simulink model "Controller"  (R2018b)
settings: configuration reference "control_config" (kept outside this file)
values from neighbouring files (symbols this model uses):
  CONTROL_EXPORT = Simulink.Parameter(CONTROL_EXPORT_VALUE)    [controller_model_init.m]
  CONTROL_PARAM = Simulink.Parameter(CONTROL_PARAM_VALUE)    [controller_model_init.m]
undefined symbols (not defined in the file or in its folder): actuator_cmd, CONTROL_CONST, ControlMode, DiscIntNeverNeededParam, timestamp, VehicleStatus
libraries: simulink x27, FMT_Model_Lib x7
(part 1 of 3)
settings Model: Creator=jc  LastModifiedBy=zouji
settings ConfigSetRef: SourceLocation=Base Workspace

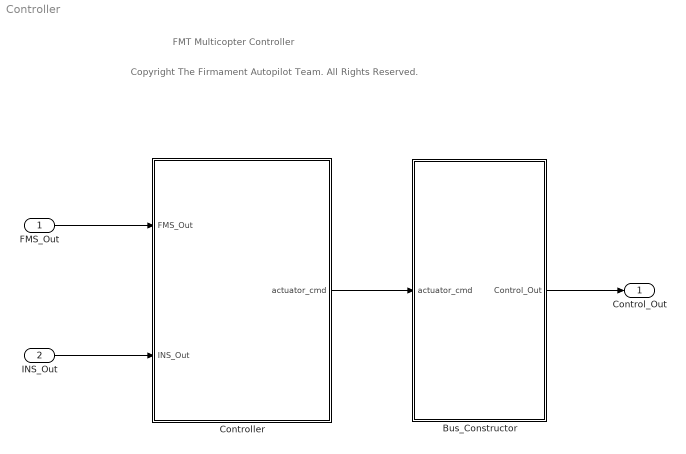
== system Controller ==
  note: Copyright The Firmament Autopilot Team. All Rights Reserved.
  note: FMT Multicopter Controller
  FMS_Out : Inport  OutDataTypeStr=Bus: FMS_Out_Bus
  INS_Out : Inport  Port=2  OutDataTypeStr=Bus: INS_Out_Bus
  Bus_Constructor : Subsystem
  Controller : Subsystem
  Control_Out : Outport  OutDataTypeStr=Bus: Control_Out_Bus
  wires:
  FMS_Out/1 -> Controller/1(FMS_Out)
  INS_Out/1 -> Controller/2(INS_Out)
  Controller/1(actuator_cmd) -> Bus_Constructor/1(actuator_cmd)
  Bus_Constructor/1(Control_Out) -> Control_Out/1

== system Controller/Bus_Constructor ==
  actuator_cmd : Inport
  Bus Assignment : BusAssignment  AssignedSignals=actuator_cmd,timestamp
  Constant : Constant  Value=0  OutDataTypeStr=Bus: Control_Out_Bus
  timestamp : Subsystem  mask{sample_time=CONTROL_EXPORT.period}
      mask prompts: sample_time "sample time (ms)"
  Control_Out : Outport
  wires:
  actuator_cmd/1 -> Bus Assignment/2
  Constant/1 -> Bus Assignment/1
  Bus Assignment/1 -> Control_Out/1
  timestamp/1(timestamp_ms) -> Bus Assignment/3

== system Controller/Controller ==
  FMS_Out : Inport
  INS_Out : Inport  Port=2
  Control_Allocation : Subsystem  Variant=on
      settings: GeneratePreprocessorConditionals=on
  Horizontal_Control : Subsystem
  Vertical_Control : Subsystem
  actuator_cmd : Outport
  wires:
  FMS_Out/1 -> Vertical_Control/1(FMS_Out), Control_Allocation/1(FMS_Out), Horizontal_Control/1(FMS_Out)
  INS_Out/1 -> Vertical_Control/2(INS_Out), Horizontal_Control/2(INS_Out)
  Horizontal_Control/1(torque_cmd_B) -> Control_Allocation/2(torque_cmd_B)  "torque_cmd_B"
  Vertical_Control/1(throttle_cmd_B) -> Control_Allocation/3(throttle_cmd_B)  "throttle_cmd_B"
  Control_Allocation/1(actuator_cmd) -> actuator_cmd/1

== system Controller/Bus_Constructor/timestamp ==
  Constant : Constant  Value=sample_time
  Data Type Conversion : DataTypeConversion  OutDataTypeStr=uint32
  Discrete-Time Integrator : DiscreteIntegrator  IntegratorMethod=Accumulation: Forward Euler  SampleTime=-1  ICPrevOutput=DiscIntNeverNeededParam  ICPrevScaledInput=DiscIntNeverNeededParam
  timestamp_ms : Outport
  wires:
  Discrete-Time Integrator/1 -> Data Type Conversion/1
  Constant/1 -> Discrete-Time Integrator/1
  Data Type Conversion/1 -> timestamp_ms/1

== system Controller/Controller/Control_Allocation ==
  note: 1) Add Subsystem or Model blocks as valid variant choices.
      | 2) You cannot connect blocks at this level. At simulation, connectivity is automatically
      | determined, based on the active variant and port name matching.
  FMS_Out : Inport
  torque_cmd_B : Inport  Port=2
  throttle_cmd_B : Inport  Port=3
  Coxial_Hexacopter_x : Subsystem  TreatAsAtomicUnit=on  VariantControl=AIRFRAME==6
      mask Display: image('.\figures\cox_hexa_x.png');
  Coxial_Quadcopter_x : Subsystem  TreatAsAtomicUnit=on  VariantControl=AIRFRAME==3
      mask Display: image('.\figures\cox_quad_x.png');
  Hexacopter_+ : Subsystem  TreatAsAtomicUnit=on  VariantControl=AIRFRAME==5
      mask Display: image('.\figures\hexa_+.png');
  Hexacopter_x : Subsystem  TreatAsAtomicUnit=on  VariantControl=AIRFRAME==4
      mask Display: image('.\figures\hexa_x.png');
  Octocopter_+ : Subsystem  TreatAsAtomicUnit=on  VariantControl=AIRFRAME==8
      mask Display: image('.\figures\octo_+.png');
  Octocopter_x : Subsystem  TreatAsAtomicUnit=on  VariantControl=AIRFRAME==7
      mask Display: image('.\figures\octo_x.png');
  Quadcopter_+ : Subsystem  TreatAsAtomicUnit=on  VariantControl=AIRFRAME==2
      mask Display: image('.\figures\quad_+.png');
  Quadcopter_x : Subsystem  TreatAsAtomicUnit=on  VariantControl=AIRFRAME==1
      mask Display: image('.\figures\quad_x.png');
  actuator_cmd : Outport

== system Controller/Controller/Horizontal_Control ==
  FMS_Out : Inport
  INS_Out : Inport  Port=2
  Attitude_Controller : Subsystem
  Bus Selector : BusSelector  OutputSignals=ctrl_mode
  Compare To Constant : simulink/Logic and Bit Operations/Compare To Constant  relop=>=  const=uint8(ControlMode.POSCTL)  OutDataTypeStr=boolean
  Velocity_Controller : Subsystem
  torque_cmd_B : Outport
  wires:
  Attitude_Controller/1(rate_dot_cmd_B) -> torque_cmd_B/1
  FMS_Out/1 -> Bus Selector/1, Attitude_Controller/2(FMS_Out), Velocity_Controller/1(FMS_Out)
  INS_Out/1 -> Velocity_Controller/2(INS_Out), Attitude_Controller/3(INS_Out)
  Velocity_Controller/1(att_cmd_B_rad) -> Attitude_Controller/1(att_cmd_B_rad)
  Bus Selector/1 -> Compare To Constant/1  "<ctrl_mode>"
  Compare To Constant/1 -> Velocity_Controller/Enable

== system Controller/Controller/Vertical_Control ==
  FMS_Out : Inport
  INS_Out : Inport  Port=2
  Bus Selector : BusSelector  OutputSignals=ctrl_mode
  Bus Selector1 : BusSelector  OutputSignals=status
  Compare To Constant : simulink/Logic and Bit Operations/Compare To Constant  relop=>=  const=uint8(ControlMode.ALTCTL)  OutDataTypeStr=boolean
  Delay : Delay  DelayLength=1  InitialCondition=uint8(VehicleStatus.Disarm)
  Signal_Select : Subsystem
  Veloxity_Z_Controller : Subsystem
  throttle_cmd_B : Outport
  wires:
  INS_Out/1 -> Veloxity_Z_Controller/3(INS_Out)
  Veloxity_Z_Controller/1(throttle_cmd) -> Signal_Select/2(throttle_cmd_in)
  FMS_Out/1 -> Bus Selector1/1, Bus Selector/1, Signal_Select/1(FMS_Out), Veloxity_Z_Controller/1(FMS_Out)
  Bus Selector/1 -> Compare To Constant/1  "<ctrl_mode>"
  Compare To Constant/1 -> Veloxity_Z_Controller/Enable
  Bus Selector1/1 -> Delay/1  "<status>"
  Delay/1 -> Veloxity_Z_Controller/2(prev_status)
  Signal_Select/1(throttle_cmd) -> throttle_cmd_B/1

== system Controller/Controller/Control_Allocation/Coxial_Hexacopter_x ==
  FMS_Out : Inport
  torque_cmd_B : Inport  Port=2
  throttle_cmd_B : Inport  Port=3
  Bus Selector : BusSelector  OutputSignals=status
  Effective_Matrix : Constant  Value=[-1/2 0 -1/2;1/2 0 1/2;(sqrt(2)-1)/2 sqrt(6)/6 -1/2;-(sqrt(2)-1)/2 -sqrt(6)/6 1/2;-(sqrt(2)-1)/2 sqrt(6)/6 1/2;(sqrt(2)-1)/2 -sqrt(6)/6 -1/2;-1/2 0 1/2;1/2 0 -1/2;(sqrt(2)-1)/2 sqrt(6)/6 1/2;-(sqrt(2)-1)/2 -sqrt(6)/6 -1/2;-(sqrt(2)-1)/2 sqrt(6)/6 -1/2;(sqrt(2)-1)/2 -sqrt(6)/6 1/2]  OutDataTypeStr=single
  Roll_Pitch_Remix : Subsystem  mask{up_lim=0.9, lo_lim=0.1}
      mask prompts: up_lim "Upper Limit"; lo_lim "Lower Limit"
  Saturation1 : Saturate  UpperLimit=1  LowerLimit=-1
  Saturation2 : Saturate  UpperLimit=1  LowerLimit=0
  Yaw_Remix : Subsystem  mask{up_lim=0.9, lo_lim=0.1}
      mask prompts: up_lim "Upper Limit"; lo_lim "Lower Limit"
  actuator_cmd_routing : Subsystem
  actuator_cmd : Outport
  wires:
  Effective_Matrix/1 -> Roll_Pitch_Remix/1(Effective_Matrix), Yaw_Remix/1(Effective_Matrix)
  throttle_cmd_B/1 -> Saturation2/1
  torque_cmd_B/1 -> Saturation1/1
  Bus Selector/1 -> actuator_cmd_routing/2(status)  "<status>"
  Saturation1/1 -> Yaw_Remix/2(torque_cmd), Roll_Pitch_Remix/2(torque_cmd)
  Roll_Pitch_Remix/1(pq_remix_throttle) -> Yaw_Remix/3(pq_remix)
  Yaw_Remix/1(pqr_remix_throttle) -> actuator_cmd_routing/1(throttle_cmd)
  actuator_cmd_routing/1(actuator_cmd) -> actuator_cmd/1
  FMS_Out/1 -> Bus Selector/1
  Saturation2/1 -> Roll_Pitch_Remix/3(throttle_cmd)

== system Controller/Controller/Control_Allocation/Coxial_Quadcopter_x ==
  FMS_Out : Inport
  torque_cmd_B : Inport  Port=2
  throttle_cmd_B : Inport  Port=3
  Bus Selector : BusSelector  OutputSignals=status
  Effective_Matrix : Constant  Value=[-1/2 1/2 1/2;1/2 1/2 -1/2;1/2 -1/2 1/2;-1/2 -1/2 -1/2;1/2 1/2 1/2;-1/2 1/2 -1/2;-1/2 -1/2 1/2;1/2 -1/2 -1/2]  OutDataTypeStr=single
  Roll_Pitch_Remix : Subsystem  mask{up_lim=0.9, lo_lim=0.1}
      mask prompts: up_lim "Upper Limit"; lo_lim "Lower Limit"
  Saturation1 : Saturate  UpperLimit=1  LowerLimit=-1
  Saturation2 : Saturate  UpperLimit=1  LowerLimit=0
  Yaw_Remix : Subsystem  mask{up_lim=0.9, lo_lim=0.1}
      mask prompts: up_lim "Upper Limit"; lo_lim "Lower Limit"
  actuator_cmd_routing : Subsystem
  actuator_cmd : Outport
  wires:
  Roll_Pitch_Remix/1(pq_remix_throttle) -> Yaw_Remix/3(pq_remix)
  Effective_Matrix/1 -> Yaw_Remix/1(Effective_Matrix), Roll_Pitch_Remix/1(Effective_Matrix)
  torque_cmd_B/1 -> Saturation1/1
  throttle_cmd_B/1 -> Saturation2/1
  FMS_Out/1 -> Bus Selector/1
  Saturation1/1 -> Yaw_Remix/2(torque_cmd), Roll_Pitch_Remix/2(torque_cmd)
  Saturation2/1 -> Roll_Pitch_Remix/3(throttle_cmd)
  Yaw_Remix/1(pqr_remix_throttle) -> actuator_cmd_routing/1(throttle_cmd)
  actuator_cmd_routing/1(actuator_cmd) -> actuator_cmd/1
  Bus Selector/1 -> actuator_cmd_routing/2(status)  "<status>"

== system Controller/Controller/Control_Allocation/Hexacopter_+ ==
  FMS_Out : Inport
  torque_cmd_B : Inport  Port=2
  throttle_cmd_B : Inport  Port=3
  Bus Selector : BusSelector  OutputSignals=status
  Effective_Matrix : Constant  Value=[0 1/2 -1/2;0 -1/2 1/2;sqrt(6)/6 -(sqrt(2)-1)/2 -1/2;-sqrt(6)/6 (sqrt(2)-1)/2 1/2;sqrt(6)/6 (sqrt(2)-1)/2 1/2;-sqrt(6)/6 -(sqrt(2)-1)/2 -1/2]  OutDataTypeStr=single
  Roll_Pitch_Remix : Subsystem  mask{up_lim=0.9, lo_lim=0.1}
      mask prompts: up_lim "Upper Limit"; lo_lim "Lower Limit"
  Saturation1 : Saturate  UpperLimit=1  LowerLimit=-1
  Saturation2 : Saturate  UpperLimit=1  LowerLimit=0
  Yaw_Remix : Subsystem  mask{up_lim=0.9, lo_lim=0.1}
      mask prompts: up_lim "Upper Limit"; lo_lim "Lower Limit"
  actuator_cmd_routing : Subsystem
  actuator_cmd : Outport
  wires:
  Saturation1/1 -> Yaw_Remix/2(torque_cmd), Roll_Pitch_Remix/2(torque_cmd)
  Effective_Matrix/1 -> Roll_Pitch_Remix/1(Effective_Matrix), Yaw_Remix/1(Effective_Matrix)
  Saturation2/1 -> Roll_Pitch_Remix/3(throttle_cmd)
  throttle_cmd_B/1 -> Saturation2/1
  actuator_cmd_routing/1(actuator_cmd) -> actuator_cmd/1
  Bus Selector/1 -> actuator_cmd_routing/2(status)  "<status>"
  Roll_Pitch_Remix/1(pq_remix_throttle) -> Yaw_Remix/3(pq_remix)
  FMS_Out/1 -> Bus Selector/1
  Yaw_Remix/1(pqr_remix_throttle) -> actuator_cmd_routing/1(throttle_cmd)
  torque_cmd_B/1 -> Saturation1/1

== system Controller/Controller/Control_Allocation/Hexacopter_x ==
  FMS_Out : Inport
  torque_cmd_B : Inport  Port=2
  throttle_cmd_B : Inport  Port=3
  Bus Selector : BusSelector  OutputSignals=status
  Effective_Matrix : Constant  Value=[-1/2 0 -1/2;1/2 0 1/2;(sqrt(2)-1)/2 sqrt(6)/6 -1/2;-(sqrt(2)-1)/2 -sqrt(6)/6 1/2;-(sqrt(2)-1)/2 sqrt(6)/6 1/2;(sqrt(2)-1)/2 -sqrt(6)/6 -1/2]  OutDataTypeStr=single
  Roll_Pitch_Remix : Subsystem  mask{up_lim=0.9, lo_lim=0.1}
      mask prompts: up_lim "Upper Limit"; lo_lim "Lower Limit"
  Saturation1 : Saturate  UpperLimit=1  LowerLimit=-1
  Saturation2 : Saturate  UpperLimit=1  LowerLimit=0
  Yaw_Remix : Subsystem  mask{up_lim=0.9, lo_lim=0.1}
      mask prompts: up_lim "Upper Limit"; lo_lim "Lower Limit"
  actuator_cmd_routing : Subsystem
  actuator_cmd : Outport
  wires:
  throttle_cmd_B/1 -> Saturation2/1
  Saturation1/1 -> Yaw_Remix/2(torque_cmd), Roll_Pitch_Remix/2(torque_cmd)
  FMS_Out/1 -> Bus Selector/1
  Bus Selector/1 -> actuator_cmd_routing/2(status)  "<status>"
  Roll_Pitch_Remix/1(pq_remix_throttle) -> Yaw_Remix/3(pq_remix)
  Saturation2/1 -> Roll_Pitch_Remix/3(throttle_cmd)
  Yaw_Remix/1(pqr_remix_throttle) -> actuator_cmd_routing/1(throttle_cmd)
  Effective_Matrix/1 -> Yaw_Remix/1(Effective_Matrix), Roll_Pitch_Remix/1(Effective_Matrix)
  actuator_cmd_routing/1(actuator_cmd) -> actuator_cmd/1
  torque_cmd_B/1 -> Saturation1/1

== system Controller/Controller/Control_Allocation/Octocopter_+ ==
  FMS_Out : Inport
  torque_cmd_B : Inport  Port=2
  throttle_cmd_B : Inport  Port=3
  Bus Selector : BusSelector  OutputSignals=status
  Effective_Matrix : Constant  Value=[0 0.5 -0.5;0 -0.5 -0.5;-0.146 0.146 0.5;-0.146 -0.146 0.5;0.146 0.146 0.5;0.146 -0.146 0.5;0.5 0 -0.5;-0.5 0 -0.5]  OutDataTypeStr=single
  Roll_Pitch_Remix : Subsystem  mask{up_lim=0.9, lo_lim=0.1}
      mask prompts: up_lim "Upper Limit"; lo_lim "Lower Limit"
  Saturation1 : Saturate  UpperLimit=1  LowerLimit=-1
  Saturation2 : Saturate  UpperLimit=1  LowerLimit=0
  Yaw_Remix : Subsystem  mask{up_lim=0.9, lo_lim=0.1}
      mask prompts: up_lim "Upper Limit"; lo_lim "Lower Limit"
  actuator_cmd_routing : Subsystem
  actuator_cmd : Outport
  wires:
  throttle_cmd_B/1 -> Saturation2/1
  Saturation2/1 -> Roll_Pitch_Remix/3(throttle_cmd)
  actuator_cmd_routing/1(actuator_cmd) -> actuator_cmd/1
  Roll_Pitch_Remix/1(pq_remix_throttle) -> Yaw_Remix/3(pq_remix)
  Effective_Matrix/1 -> Roll_Pitch_Remix/1(Effective_Matrix), Yaw_Remix/1(Effective_Matrix)
  Yaw_Remix/1(pqr_remix_throttle) -> actuator_cmd_routing/1(throttle_cmd)
  Bus Selector/1 -> actuator_cmd_routing/2(status)  "<status>"
  Saturation1/1 -> Yaw_Remix/2(torque_cmd), Roll_Pitch_Remix/2(torque_cmd)
  torque_cmd_B/1 -> Saturation1/1
  FMS_Out/1 -> Bus Selector/1

== system Controller/Controller/Control_Allocation/Octocopter_x ==
  FMS_Out : Inport
  torque_cmd_B : Inport  Port=2
  throttle_cmd_B : Inport  Port=3
  Bus Selector : BusSelector  OutputSignals=status
  Effective_Matrix : Constant  Value=[-0.15 0.5 -0.5;0.15 -0.5 -0.5;-0.5 0.15 0.5;-0.15 -0.5 0.5;0.15 0.5 0.5;0.5 -0.15 0.5;0.5 0.15 -0.5;-0.5 -0.15 -0.5]  OutDataTypeStr=single
  Roll_Pitch_Remix : Subsystem  mask{up_lim=0.9, lo_lim=0.1}
      mask prompts: up_lim "Upper Limit"; lo_lim "Lower Limit"
  Saturation1 : Saturate  UpperLimit=1  LowerLimit=-1
  Saturation2 : Saturate  UpperLimit=1  LowerLimit=0
  Yaw_Remix : Subsystem  mask{up_lim=0.9, lo_lim=0.1}
      mask prompts: up_lim "Upper Limit"; lo_lim "Lower Limit"
  actuator_cmd_routing : Subsystem
  actuator_cmd : Outport
  wires:
  torque_cmd_B/1 -> Saturation1/1
  Bus Selector/1 -> actuator_cmd_routing/2(status)  "<status>"
  Yaw_Remix/1(pqr_remix_throttle) -> actuator_cmd_routing/1(throttle_cmd)
  Saturation2/1 -> Roll_Pitch_Remix/3(throttle_cmd)
  Saturation1/1 -> Yaw_Remix/2(torque_cmd), Roll_Pitch_Remix/2(torque_cmd)
  FMS_Out/1 -> Bus Selector/1
  Roll_Pitch_Remix/1(pq_remix_throttle) -> Yaw_Remix/3(pq_remix)
  actuator_cmd_routing/1(actuator_cmd) -> actuator_cmd/1
  throttle_cmd_B/1 -> Saturation2/1
  Effective_Matrix/1 -> Roll_Pitch_Remix/1(Effective_Matrix), Yaw_Remix/1(Effective_Matrix)

== system Controller/Controller/Control_Allocation/Quadcopter_+ ==
  FMS_Out : Inport
  torque_cmd_B : Inport  Port=2
  throttle_cmd_B : Inport  Port=3
  Bus Selector : BusSelector  OutputSignals=status
  Effective_Matrix : Constant  Value=[-1/2 0 1/2;1/2 0 1/2;0 1/2 -1/2;0 -1/2 -1/2]  OutDataTypeStr=single
  Roll_Pitch_Remix : Subsystem  mask{up_lim=0.9, lo_lim=0.1}
      mask prompts: up_lim "Upper Limit"; lo_lim "Lower Limit"
  Saturation1 : Saturate  UpperLimit=1  LowerLimit=-1
  Saturation2 : Saturate  UpperLimit=1  LowerLimit=0
  Yaw_Remix : Subsystem  mask{up_lim=0.9, lo_lim=0.1}
      mask prompts: up_lim "Upper Limit"; lo_lim "Lower Limit"
  actuator_cmd_routing : Subsystem
  actuator_cmd : Outport
  wires:
  Effective_Matrix/1 -> Yaw_Remix/1(Effective_Matrix), Roll_Pitch_Remix/1(Effective_Matrix)
  Roll_Pitch_Remix/1(pq_remix_throttle) -> Yaw_Remix/3(pq_remix)
  torque_cmd_B/1 -> Saturation1/1
  Yaw_Remix/1(pqr_remix_throttle) -> actuator_cmd_routing/1(throttle_cmd)
  Saturation1/1 -> Yaw_Remix/2(torque_cmd), Roll_Pitch_Remix/2(torque_cmd)
  actuator_cmd_routing/1(actuator_cmd) -> actuator_cmd/1
  Saturation2/1 -> Roll_Pitch_Remix/3(throttle_cmd)
  throttle_cmd_B/1 -> Saturation2/1
  FMS_Out/1 -> Bus Selector/1
  Bus Selector/1 -> actuator_cmd_routing/2(status)  "<status>"

== system Controller/Controller/Control_Allocation/Quadcopter_x ==
  FMS_Out : Inport
  torque_cmd_B : Inport  Port=2
  throttle_cmd_B : Inport  Port=3
  Bus Selector : BusSelector  OutputSignals=status
  Effective_Matrix : Constant  Value=[-1/2 1/2 1/2;1/2 -1/2 1/2;1/2 1/2 -1/2;-1/2 -1/2 -1/2]  OutDataTypeStr=single
  Roll_Pitch_Remix : Subsystem  mask{up_lim=0.9, lo_lim=0.1}
      mask prompts: up_lim "Upper Limit"; lo_lim "Lower Limit"
  Saturation1 : Saturate  UpperLimit=1  LowerLimit=-1
  Saturation2 : Saturate  UpperLimit=1  LowerLimit=0
  Yaw_Remix : Subsystem  mask{up_lim=0.9, lo_lim=0.1}
      mask prompts: up_lim "Upper Limit"; lo_lim "Lower Limit"
  actuator_cmd_routing : Subsystem
  actuator_cmd : Outport
  wires:
  Effective_Matrix/1 -> Yaw_Remix/1(Effective_Matrix), Roll_Pitch_Remix/1(Effective_Matrix)
  Saturation1/1 -> Yaw_Remix/2(torque_cmd), Roll_Pitch_Remix/2(torque_cmd)
  Roll_Pitch_Remix/1(pq_remix_throttle) -> Yaw_Remix/3(pq_remix)
  Bus Selector/1 -> actuator_cmd_routing/2(status)  "<status>"
  torque_cmd_B/1 -> Saturation1/1
  Yaw_Remix/1(pqr_remix_throttle) -> actuator_cmd_routing/1(throttle_cmd)
  throttle_cmd_B/1 -> Saturation2/1
  FMS_Out/1 -> Bus Selector/1
  actuator_cmd_routing/1(actuator_cmd) -> actuator_cmd/1
  Saturation2/1 -> Roll_Pitch_Remix/3(throttle_cmd)

== system Controller/Controller/Horizontal_Control/Attitude_Controller ==
  att_cmd_B_rad : Inport
  FMS_Out : Inport  Port=2
  INS_Out : Inport  Port=3
  Inner_Loop : Subsystem
  Outter_Loop : Subsystem
  rate_dot_cmd_B : Outport
  wires:
  INS_Out/1 -> Inner_Loop/2(INS_Out), Outter_Loop/2(INS_Out)
  FMS_Out/1 -> Inner_Loop/3(FMS_Out), Outter_Loop/3(FMS_Out)
  att_cmd_B_rad/1 -> Outter_Loop/1(att_cmd_rad)
  Outter_Loop/1(euler_rate_cmd_radPs) -> Inner_Loop/1(euler_rate_cmd_radPs)
  Inner_Loop/1(rate_dot_cmd_B) -> rate_dot_cmd_B/1

== system Controller/Controller/Horizontal_Control/Velocity_Controller ==
  FMS_Out : Inport
  INS_Out : Inport  Port=2
  Enable : EnablePort  StatesWhenEnabling=reset
  Accel_to_Attitude_CMD : Subsystem
  Bus Selector : BusSelector  OutputSignals=reset
  Error : Subsystem
  PID_Controller : Subsystem
  Signal_Select : Subsystem
  att_cmd_B_rad : Outport
  wires:
  FMS_Out/1 -> Signal_Select/2(FMS_Out), Error/2(FMS_Out), Bus Selector/1
  PID_Controller/1(accel_cmd_C) -> Signal_Select/1(acc_cmd_in)  "accel_cmd_C_mPs2"
  INS_Out/1 -> Error/1(INS_Out)
  Error/1(uv_err_C_mPs) -> PID_Controller/1(uv_err_C_mPs)
  Accel_to_Attitude_CMD/1(att_cmd_B_rad) -> att_cmd_B_rad/1
  Bus Selector/1 -> PID_Controller/2(reset)  "<reset>"
  Signal_Select/1(acc_cmd_out) -> Accel_to_Attitude_CMD/1(accel_cmd_C_mPs2)

== system Controller/Controller/Vertical_Control/Signal_Select ==
  FMS_Out : Inport
  throttle_cmd_in : Inport  Port=2
  Bias : Bias  Bias=-1
  Bus Selector1 : BusSelector  OutputSignals=throttle_cmd,ctrl_mode
  Compare To Constant : simulink/Logic and Bit Operations/Compare To Constant  relop=<=  const=uint8(ControlMode.Stabilize)  OutDataTypeStr=boolean
  Compare To Constant1 : simulink/Logic and Bit Operations/Compare To Constant  relop===  const=uint8(ControlMode.Offboard)  OutDataTypeStr=boolean
  Gain : Gain  Gain=1/1000  OutDataTypeStr=single
  Offboard_Signal_Select : Subsystem
  Switch : Switch  Criteria=u2 > Threshold
  Switch1 : Switch  Criteria=u2 > Threshold
  throttle_cmd : Outport
  wires:
  FMS_Out/1 -> Offboard_Signal_Select/1(FMS_Out), Bus Selector1/1
  Bus Selector1/1 -> Gain/1  "<throttle_cmd>"
  Bus Selector1/2 -> Compare To Constant/1, Compare To Constant1/1  "<ctrl_mode>"
  Switch/1 -> throttle_cmd/1
  Compare To Constant/1 -> Switch/2
  throttle_cmd_in/1 -> Offboard_Signal_Select/2(throttle_cmd_in), Switch1/3
  Compare To Constant1/1 -> Switch1/2
  Switch1/1 -> Switch/3
  Offboard_Signal_Select/1(throttle_cmd_out) -> Switch1/1
  Gain/1 -> Bias/1
  Bias/1 -> Switch/1

== system Controller/Controller/Vertical_Control/Veloxity_Z_Controller ==
  FMS_Out : Inport
  prev_status : Inport  Port=2
  INS_Out : Inport  Port=3
  Enable : EnablePort  StatesWhenEnabling=reset
  Boosted_Throttle : Subsystem
  Bus Selector : BusSelector  OutputSignals=reset
  Error : Subsystem
  PID_Controller : Subsystem
  Saturation : Saturate  UpperLimit=0.7  LowerLimit=0.3
  Sum : Sum  Inputs=|++
  hover_throttle : Constant  Value=CONTROL_PARAM.MC_HOVER_THRO  OutDataTypeStr=Inherit: Inherit via back propagation
  throttle_cmd : Outport
  wires:
  Saturation/1 -> throttle_cmd/1
  INS_Out/1 -> Boosted_Throttle/2(INS_Out), Error/2(INS_Out)
  Boosted_Throttle/1(boosted_thrust) -> Sum/1  "boosted_thrust"
  Error/1(az_cmd_C_mPs2) -> PID_Controller/1(az_cmd_C_mPs2)
  FMS_Out/1 -> Bus Selector/1, Error/1(FMS_Out)
  PID_Controller/1(thrust_cmd) -> Boosted_Throttle/1(thrust_cmd)
  prev_status/1 -> PID_Controller/3(prev_status)
  Bus Selector/1 -> PID_Controller/2(reset)  "<reset>"
  hover_throttle/1 -> Sum/2
  Sum/1 -> Saturation/1

== system Controller/Controller/Control_Allocation/Coxial_Hexacopter_x/Roll_Pitch_Remix ==
  Effective_Matrix : Inport
  torque_cmd : Inport  Port=2
  throttle_cmd : Inport  Port=3
  Constant : Constant  Value=up_lim  OutDataTypeStr=single
  Constant1 : Constant  Value=lo_lim  OutDataTypeStr=single
  Max : MinMax  Function=max
  Max1 : MinMax
  Multiply : Product  Multiplication=Matrix(*)  OutDataTypeStr=single
  Multiply1 : Product  OutDataTypeStr=single
  PQ_Remix : Subsystem
  Reshape : Reshape  OutputDimensionality=Column vector (2-D)
  Saturation3 : Saturate  UpperLimit=1  LowerLimit=0
  Saturation4 : Saturate  UpperLimit=1  LowerLimit=0
  Selector : Selector  InputPortWidth=3  IndexOptions=Index vector (dialog)  Indices=[1 2]  OutputSizes=1
  Sum : Sum  Inputs=|++
  Sum1 : Sum  Inputs=|++
  Sum2 : Sum  Inputs=|++
  pq_column : Selector  NumberOfDimensions=2  InputPortWidth=3  IndexOptions=Select all,Index vector (dialog)  Indices=[1:4],[1 2]  OutputSizes=1,1
  pq_remix_throttle : Outport
  wires:
  Multiply1/1 -> Sum2/1
  Multiply/1 -> Multiply1/1, Sum/1
  Constant1/1 -> PQ_Remix/4(lo_min)
  Sum/1 -> Max/1, Max1/1  "pq_premix"
  Max1/1 -> PQ_Remix/2(min)
  pq_column/1 -> Multiply/1
  Constant/1 -> PQ_Remix/3(up_lim)
  throttle_cmd/1 -> PQ_Remix/5(force_z_cmd), Sum/2, Sum1/2
  Reshape/1 -> Multiply/2
  Sum2/1 -> Saturation4/1  "pq_remix"
  Sum1/1 -> Saturation3/1
  PQ_Remix/1(roll_pitch_scale) -> Multiply1/2  "roll_pitch_scale"
  Saturation3/1 -> Sum2/2
  Selector/1 -> Reshape/1
  Saturation4/1 -> pq_remix_throttle/1
  Max/1 -> PQ_Remix/1(max)
  PQ_Remix/2(floating_throttle) -> Sum1/1  "floating_throttle"
  Effective_Matrix/1 -> pq_column/1
  torque_cmd/1 -> Selector/1

== system Controller/Controller/Control_Allocation/Coxial_Hexacopter_x/Yaw_Remix ==
  Effective_Matrix : Inport
  torque_cmd : Inport  Port=2
  pq_remix : Inport  Port=3
  Constant : Constant  Value=up_lim  OutDataTypeStr=single
  Constant1 : Constant  Value=lo_lim  OutDataTypeStr=single
  Multiply2 : Product  Multiplication=Matrix(*)  OutDataTypeStr=single
  R_Remix : MATLAB Function  TreatAsAtomicUnit=on
  Selector2 : Selector  InputPortWidth=3  IndexOptions=Index vector (dialog)  Indices=3  OutputSizes=1
  Sum3 : Sum  Inputs=|++
  Sum4 : Sum  Inputs=++|
  r_column : Selector  NumberOfDimensions=2  InputPortWidth=3  IndexOptions=Select all,Index vector (dialog)  Indices=[1:4],3  OutputSizes=1,1
  pqr_remix_throttle : Outport
  wires:
  Sum4/1 -> pqr_remix_throttle/1  "pqr_remix"
  Selector2/1 -> Multiply2/2
  Effective_Matrix/1 -> r_column/1
  torque_cmd/1 -> Selector2/1
  r_column/1 -> R_Remix/3(r_column), Multiply2/1
  Sum3/1 -> Sum4/2, R_Remix/4(motor_out)
  Multiply2/1 -> Sum3/1
  pq_remix/1 -> Sum3/2
  Constant/1 -> R_Remix/1(up_lim)
  Constant1/1 -> R_Remix/2(lo_lim)
  R_Remix/1(floating_yaw) -> Sum4/1  "floating_yaw"

== system Controller/Controller/Control_Allocation/Coxial_Hexacopter_x/actuator_cmd_routing ==
  throttle_cmd : Inport
  status : Inport  Port=2
  Constant : Constant  Value=zeros(4,1)  VectorParams1D=off  OutDataTypeStr=uint16
  Constant2 : Constant  Value=1000  OutDataTypeStr=uint32
  Data Type Conversion : DataTypeConversion  OutDataTypeStr=uint16
  Disarm : Constant  Value=ones(12,1)*1000  VectorParams1D=off  OutDataTypeStr=uint16
  Gain3 : Gain  Gain=1000  OutDataTypeStr=uint32
  Multiport Switch : MultiPortSwitch  DataPortForDefault=Additional data port  DiagnosticForDefault=None
  Mux1 : Mux  Inputs=2
  Reshape : Reshape  OutputDimensionality=Customize  OutputDimensions=[16,1]
  Saturation5 : Saturate  UpperLimit=1  LowerLimit=0
  Standby : Constant  Value=ones(12,1)*1150  VectorParams1D=off  OutDataTypeStr=uint16
  Sum5 : Sum  Inputs=|++
  actuator_cmd : Outport
  wires:
  Disarm/1 -> Multiport Switch/5, Multiport Switch/2
  Reshape/1 -> actuator_cmd/1
  Constant/1 -> Mux1/2
  Standby/1 -> Multiport Switch/3
  Mux1/1 -> Reshape/1
  status/1 -> Multiport Switch/1
  Multiport Switch/1 -> Mux1/1
  Sum5/1 -> Data Type Conversion/1
  Saturation5/1 -> Gain3/1
  Gain3/1 -> Sum5/1
  Constant2/1 -> Sum5/2
  throttle_cmd/1 -> Saturation5/1
  Data Type Conversion/1 -> Multiport Switch/4

== system Controller/Controller/Control_Allocation/Coxial_Quadcopter_x/Roll_Pitch_Remix ==
  Effective_Matrix : Inport
  torque_cmd : Inport  Port=2
  throttle_cmd : Inport  Port=3
  Constant : Constant  Value=up_lim  OutDataTypeStr=single
  Constant1 : Constant  Value=lo_lim  OutDataTypeStr=single
  Max : MinMax  Function=max
  Max1 : MinMax
  Multiply : Product  Multiplication=Matrix(*)  OutDataTypeStr=single
  Multiply1 : Product  OutDataTypeStr=single
  PQ_Remix : Subsystem
  Reshape : Reshape  OutputDimensionality=Column vector (2-D)
  Saturation3 : Saturate  UpperLimit=1  LowerLimit=0
  Saturation4 : Saturate  UpperLimit=1  LowerLimit=0
  Selector : Selector  InputPortWidth=3  IndexOptions=Index vector (dialog)  Indices=[1 2]  OutputSizes=1
  Sum : Sum  Inputs=|++
  Sum1 : Sum  Inputs=|++
  Sum2 : Sum  Inputs=|++
  pq_column : Selector  NumberOfDimensions=2  InputPortWidth=3  IndexOptions=Select all,Index vector (dialog)  Indices=[1:4],[1 2]  OutputSizes=1,1
  pq_remix_throttle : Outport
  wires:
  Multiply1/1 -> Sum2/1
  Multiply/1 -> Multiply1/1, Sum/1
  Constant1/1 -> PQ_Remix/4(lo_min)
  Sum/1 -> Max/1, Max1/1  "pq_premix"
  Max1/1 -> PQ_Remix/2(min)
  pq_column/1 -> Multiply/1
  Constant/1 -> PQ_Remix/3(up_lim)
  throttle_cmd/1 -> PQ_Remix/5(force_z_cmd), Sum/2, Sum1/2
  Reshape/1 -> Multiply/2
  Sum2/1 -> Saturation4/1  "pq_remix"
  Sum1/1 -> Saturation3/1
  PQ_Remix/1(roll_pitch_scale) -> Multiply1/2  "roll_pitch_scale"
  Saturation3/1 -> Sum2/2
  Selector/1 -> Reshape/1
  Saturation4/1 -> pq_remix_throttle/1
  Max/1 -> PQ_Remix/1(max)
  PQ_Remix/2(floating_throttle) -> Sum1/1  "floating_throttle"
  Effective_Matrix/1 -> pq_column/1
  torque_cmd/1 -> Selector/1

== system Controller/Controller/Control_Allocation/Coxial_Quadcopter_x/Yaw_Remix ==
  Effective_Matrix : Inport
  torque_cmd : Inport  Port=2
  pq_remix : Inport  Port=3
  Constant : Constant  Value=up_lim  OutDataTypeStr=single
  Constant1 : Constant  Value=lo_lim  OutDataTypeStr=single
  Multiply2 : Product  Multiplication=Matrix(*)  OutDataTypeStr=single
  R_Remix : MATLAB Function  TreatAsAtomicUnit=on
  Selector2 : Selector  InputPortWidth=3  IndexOptions=Index vector (dialog)  Indices=3  OutputSizes=1
  Sum3 : Sum  Inputs=|++
  Sum4 : Sum  Inputs=++|
  r_column : Selector  NumberOfDimensions=2  InputPortWidth=3  IndexOptions=Select all,Index vector (dialog)  Indices=[1:4],3  OutputSizes=1,1
  pqr_remix_throttle : Outport
  wires:
  Sum4/1 -> pqr_remix_throttle/1  "pqr_remix"
  Selector2/1 -> Multiply2/2
  Effective_Matrix/1 -> r_column/1
  torque_cmd/1 -> Selector2/1
  r_column/1 -> R_Remix/3(r_column), Multiply2/1
  Sum3/1 -> Sum4/2, R_Remix/4(motor_out)
  Multiply2/1 -> Sum3/1
  pq_remix/1 -> Sum3/2
  Constant/1 -> R_Remix/1(up_lim)
  Constant1/1 -> R_Remix/2(lo_lim)
  R_Remix/1(floating_yaw) -> Sum4/1  "floating_yaw"

== system Controller/Controller/Control_Allocation/Coxial_Quadcopter_x/actuator_cmd_routing ==
  throttle_cmd : Inport
  status : Inport  Port=2
  Constant : Constant  Value=zeros(8,1)  VectorParams1D=off  OutDataTypeStr=uint16
  Constant2 : Constant  Value=1000  OutDataTypeStr=uint32
  Data Type Conversion : DataTypeConversion  OutDataTypeStr=uint16
  Disarm : Constant  Value=ones(8,1)*1000  VectorParams1D=off  OutDataTypeStr=uint16
  Gain3 : Gain  Gain=1000  OutDataTypeStr=uint32
  Multiport Switch : MultiPortSwitch  DataPortForDefault=Additional data port  DiagnosticForDefault=None
  Mux1 : Mux  Inputs=2
  Reshape : Reshape  OutputDimensionality=Customize  OutputDimensions=[16,1]
  Saturation5 : Saturate  UpperLimit=1  LowerLimit=0
  Standby : Constant  Value=ones(8,1)*1150  VectorParams1D=off  OutDataTypeStr=uint16
  Sum5 : Sum  Inputs=|++
  actuator_cmd : Outport
  wires:
  Disarm/1 -> Multiport Switch/5, Multiport Switch/2
  Reshape/1 -> actuator_cmd/1
  Constant/1 -> Mux1/2
  Standby/1 -> Multiport Switch/3
  Mux1/1 -> Reshape/1
  status/1 -> Multiport Switch/1
  Multiport Switch/1 -> Mux1/1
  Sum5/1 -> Data Type Conversion/1
  Saturation5/1 -> Gain3/1
  Gain3/1 -> Sum5/1
  Constant2/1 -> Sum5/2
  throttle_cmd/1 -> Saturation5/1
  Data Type Conversion/1 -> Multiport Switch/4

== system Controller/Controller/Control_Allocation/Hexacopter_+/Roll_Pitch_Remix ==
  Effective_Matrix : Inport
  torque_cmd : Inport  Port=2
  throttle_cmd : Inport  Port=3
  Constant : Constant  Value=up_lim  OutDataTypeStr=single
  Constant1 : Constant  Value=lo_lim  OutDataTypeStr=single
  Max : MinMax  Function=max
  Max1 : MinMax
  Multiply : Product  Multiplication=Matrix(*)  OutDataTypeStr=single
  Multiply1 : Product  OutDataTypeStr=single
  PQ_Remix : Subsystem
  Reshape : Reshape  OutputDimensionality=Column vector (2-D)
  Saturation3 : Saturate  UpperLimit=1  LowerLimit=0
  Saturation4 : Saturate  UpperLimit=1  LowerLimit=0
  Selector : Selector  InputPortWidth=3  IndexOptions=Index vector (dialog)  Indices=[1 2]  OutputSizes=1
  Sum : Sum  Inputs=|++
  Sum1 : Sum  Inputs=|++
  Sum2 : Sum  Inputs=|++
  pq_column : Selector  NumberOfDimensions=2  InputPortWidth=3  IndexOptions=Select all,Index vector (dialog)  Indices=[1:4],[1 2]  OutputSizes=1,1
  pq_remix_throttle : Outport
  wires:
  Multiply1/1 -> Sum2/1
  Multiply/1 -> Multiply1/1, Sum/1
  Constant1/1 -> PQ_Remix/4(lo_min)
  Sum/1 -> Max/1, Max1/1  "pq_premix"
  Max1/1 -> PQ_Remix/2(min)
  pq_column/1 -> Multiply/1
  Constant/1 -> PQ_Remix/3(up_lim)
  throttle_cmd/1 -> PQ_Remix/5(force_z_cmd), Sum/2, Sum1/2
  Reshape/1 -> Multiply/2
  Sum2/1 -> Saturation4/1  "pq_remix"
  Sum1/1 -> Saturation3/1
  PQ_Remix/1(roll_pitch_scale) -> Multiply1/2  "roll_pitch_scale"
  Saturation3/1 -> Sum2/2
  Selector/1 -> Reshape/1
  Saturation4/1 -> pq_remix_throttle/1
  Max/1 -> PQ_Remix/1(max)
  PQ_Remix/2(floating_throttle) -> Sum1/1  "floating_throttle"
  Effective_Matrix/1 -> pq_column/1
  torque_cmd/1 -> Selector/1

== system Controller/Controller/Control_Allocation/Hexacopter_+/Yaw_Remix ==
  Effective_Matrix : Inport
  torque_cmd : Inport  Port=2
  pq_remix : Inport  Port=3
  Constant : Constant  Value=up_lim  OutDataTypeStr=single
  Constant1 : Constant  Value=lo_lim  OutDataTypeStr=single
  Multiply2 : Product  Multiplication=Matrix(*)  OutDataTypeStr=single
  R_Remix : MATLAB Function  TreatAsAtomicUnit=on
  Selector2 : Selector  InputPortWidth=3  IndexOptions=Index vector (dialog)  Indices=3  OutputSizes=1
  Sum3 : Sum  Inputs=|++
  Sum4 : Sum  Inputs=++|
  r_column : Selector  NumberOfDimensions=2  InputPortWidth=3  IndexOptions=Select all,Index vector (dialog)  Indices=[1:4],3  OutputSizes=1,1
  pqr_remix_throttle : Outport
  wires:
  Sum4/1 -> pqr_remix_throttle/1  "pqr_remix"
  Selector2/1 -> Multiply2/2
  Effective_Matrix/1 -> r_column/1
  torque_cmd/1 -> Selector2/1
  r_column/1 -> R_Remix/3(r_column), Multiply2/1
  Sum3/1 -> Sum4/2, R_Remix/4(motor_out)
  Multiply2/1 -> Sum3/1
  pq_remix/1 -> Sum3/2
  Constant/1 -> R_Remix/1(up_lim)
  Constant1/1 -> R_Remix/2(lo_lim)
  R_Remix/1(floating_yaw) -> Sum4/1  "floating_yaw"

== system Controller/Controller/Control_Allocation/Hexacopter_+/actuator_cmd_routing ==
  throttle_cmd : Inport
  status : Inport  Port=2
  Constant : Constant  Value=zeros(10,1)  VectorParams1D=off  OutDataTypeStr=uint16
  Constant2 : Constant  Value=1000  OutDataTypeStr=uint32
  Data Type Conversion : DataTypeConversion  OutDataTypeStr=uint16
  Disarm : Constant  Value=ones(6,1)*1000  VectorParams1D=off  OutDataTypeStr=uint16
  Gain3 : Gain  Gain=1000  OutDataTypeStr=uint32
  Multiport Switch : MultiPortSwitch  DataPortForDefault=Additional data port  DiagnosticForDefault=None
  Mux1 : Mux  Inputs=2
  Reshape : Reshape  OutputDimensionality=Customize  OutputDimensions=[16,1]
  Saturation5 : Saturate  UpperLimit=1  LowerLimit=0
  Standby : Constant  Value=ones(6,1)*1150  VectorParams1D=off  OutDataTypeStr=uint16
  Sum5 : Sum  Inputs=|++
  actuator_cmd : Outport
  wires:
  Disarm/1 -> Multiport Switch/5, Multiport Switch/2
  Reshape/1 -> actuator_cmd/1
  Constant/1 -> Mux1/2
  Standby/1 -> Multiport Switch/3
  Mux1/1 -> Reshape/1
  status/1 -> Multiport Switch/1
  Multiport Switch/1 -> Mux1/1
  Sum5/1 -> Data Type Conversion/1
  Saturation5/1 -> Gain3/1
  Gain3/1 -> Sum5/1
  Constant2/1 -> Sum5/2
  throttle_cmd/1 -> Saturation5/1
  Data Type Conversion/1 -> Multiport Switch/4

== system Controller/Controller/Control_Allocation/Hexacopter_x/Roll_Pitch_Remix ==
  Effective_Matrix : Inport
  torque_cmd : Inport  Port=2
  throttle_cmd : Inport  Port=3
  Constant : Constant  Value=up_lim  OutDataTypeStr=single
  Constant1 : Constant  Value=lo_lim  OutDataTypeStr=single
  Max : MinMax  Function=max
  Max1 : MinMax
  Multiply : Product  Multiplication=Matrix(*)  OutDataTypeStr=single
  Multiply1 : Product  OutDataTypeStr=single
  PQ_Remix : Subsystem
  Reshape : Reshape  OutputDimensionality=Column vector (2-D)
  Saturation3 : Saturate  UpperLimit=1  LowerLimit=0
  Saturation4 : Saturate  UpperLimit=1  LowerLimit=0
  Selector : Selector  InputPortWidth=3  IndexOptions=Index vector (dialog)  Indices=[1 2]  OutputSizes=1
  Sum : Sum  Inputs=|++
  Sum1 : Sum  Inputs=|++
  Sum2 : Sum  Inputs=|++
  pq_column : Selector  NumberOfDimensions=2  InputPortWidth=3  IndexOptions=Select all,Index vector (dialog)  Indices=[1:4],[1 2]  OutputSizes=1,1
  pq_remix_throttle : Outport
  wires:
  Multiply1/1 -> Sum2/1
  Multiply/1 -> Multiply1/1, Sum/1
  Constant1/1 -> PQ_Remix/4(lo_min)
  Sum/1 -> Max/1, Max1/1  "pq_premix"
  Max1/1 -> PQ_Remix/2(min)
  pq_column/1 -> Multiply/1
  Constant/1 -> PQ_Remix/3(up_lim)
  throttle_cmd/1 -> PQ_Remix/5(force_z_cmd), Sum/2, Sum1/2
  Reshape/1 -> Multiply/2
  Sum2/1 -> Saturation4/1  "pq_remix"
  Sum1/1 -> Saturation3/1
  PQ_Remix/1(roll_pitch_scale) -> Multiply1/2  "roll_pitch_scale"
  Saturation3/1 -> Sum2/2
  Selector/1 -> Reshape/1
  Saturation4/1 -> pq_remix_throttle/1
  Max/1 -> PQ_Remix/1(max)
  PQ_Remix/2(floating_throttle) -> Sum1/1  "floating_throttle"
  Effective_Matrix/1 -> pq_column/1
  torque_cmd/1 -> Selector/1

== system Controller/Controller/Control_Allocation/Hexacopter_x/Yaw_Remix ==
  Effective_Matrix : Inport
  torque_cmd : Inport  Port=2
  pq_remix : Inport  Port=3
  Constant : Constant  Value=up_lim  OutDataTypeStr=single
  Constant1 : Constant  Value=lo_lim  OutDataTypeStr=single
  Multiply2 : Product  Multiplication=Matrix(*)  OutDataTypeStr=single
  R_Remix : MATLAB Function  TreatAsAtomicUnit=on
  Selector2 : Selector  InputPortWidth=3  IndexOptions=Index vector (dialog)  Indices=3  OutputSizes=1
  Sum3 : Sum  Inputs=|++
  Sum4 : Sum  Inputs=++|
  r_column : Selector  NumberOfDimensions=2  InputPortWidth=3  IndexOptions=Select all,Index vector (dialog)  Indices=[1:4],3  OutputSizes=1,1
  pqr_remix_throttle : Outport
  wires:
  Sum4/1 -> pqr_remix_throttle/1  "pqr_remix"
  Selector2/1 -> Multiply2/2
  Effective_Matrix/1 -> r_column/1
  torque_cmd/1 -> Selector2/1
  r_column/1 -> R_Remix/3(r_column), Multiply2/1
  Sum3/1 -> Sum4/2, R_Remix/4(motor_out)
  Multiply2/1 -> Sum3/1
  pq_remix/1 -> Sum3/2
  Constant/1 -> R_Remix/1(up_lim)
  Constant1/1 -> R_Remix/2(lo_lim)
  R_Remix/1(floating_yaw) -> Sum4/1  "floating_yaw"

== system Controller/Controller/Control_Allocation/Hexacopter_x/actuator_cmd_routing ==
  throttle_cmd : Inport
  status : Inport  Port=2
  Constant : Constant  Value=zeros(10,1)  VectorParams1D=off  OutDataTypeStr=uint16
  Constant2 : Constant  Value=1000  OutDataTypeStr=uint32
  Data Type Conversion : DataTypeConversion  OutDataTypeStr=uint16
  Disarm : Constant  Value=ones(6,1)*1000  VectorParams1D=off  OutDataTypeStr=uint16
  Gain3 : Gain  Gain=1000  OutDataTypeStr=uint32
  Multiport Switch : MultiPortSwitch  DataPortForDefault=Additional data port  DiagnosticForDefault=None
  Mux1 : Mux  Inputs=2
  Reshape : Reshape  OutputDimensionality=Customize  OutputDimensions=[16,1]
  Saturation5 : Saturate  UpperLimit=1  LowerLimit=0
  Standby : Constant  Value=ones(6,1)*1150  VectorParams1D=off  OutDataTypeStr=uint16
  Sum5 : Sum  Inputs=|++
  actuator_cmd : Outport
  wires:
  Disarm/1 -> Multiport Switch/5, Multiport Switch/2
  Reshape/1 -> actuator_cmd/1
  Constant/1 -> Mux1/2
  Standby/1 -> Multiport Switch/3
  Mux1/1 -> Reshape/1
  status/1 -> Multiport Switch/1
  Multiport Switch/1 -> Mux1/1
  Sum5/1 -> Data Type Conversion/1
  Saturation5/1 -> Gain3/1
  Gain3/1 -> Sum5/1
  Constant2/1 -> Sum5/2
  throttle_cmd/1 -> Saturation5/1
  Data Type Conversion/1 -> Multiport Switch/4

== system Controller/Controller/Control_Allocation/Octocopter_+/Roll_Pitch_Remix ==
  Effective_Matrix : Inport
  torque_cmd : Inport  Port=2
  throttle_cmd : Inport  Port=3
  Constant : Constant  Value=up_lim  OutDataTypeStr=single
  Constant1 : Constant  Value=lo_lim  OutDataTypeStr=single
  Max : MinMax  Function=max
  Max1 : MinMax
  Multiply : Product  Multiplication=Matrix(*)  OutDataTypeStr=single
  Multiply1 : Product  OutDataTypeStr=single
  PQ_Remix : Subsystem
  Reshape : Reshape  OutputDimensionality=Column vector (2-D)
  Saturation3 : Saturate  UpperLimit=1  LowerLimit=0
  Saturation4 : Saturate  UpperLimit=1  LowerLimit=0
  Selector : Selector  InputPortWidth=3  IndexOptions=Index vector (dialog)  Indices=[1 2]  OutputSizes=1
  Sum : Sum  Inputs=|++
  Sum1 : Sum  Inputs=|++
  Sum2 : Sum  Inputs=|++
  pq_column : Selector  NumberOfDimensions=2  InputPortWidth=3  IndexOptions=Select all,Index vector (dialog)  Indices=[1:4],[1 2]  OutputSizes=1,1
  pq_remix_throttle : Outport
  wires:
  Multiply1/1 -> Sum2/1
  Multiply/1 -> Multiply1/1, Sum/1
  Constant1/1 -> PQ_Remix/4(lo_min)
  Sum/1 -> Max/1, Max1/1  "pq_premix"
  Max1/1 -> PQ_Remix/2(min)
  pq_column/1 -> Multiply/1
  Constant/1 -> PQ_Remix/3(up_lim)
  throttle_cmd/1 -> PQ_Remix/5(force_z_cmd), Sum/2, Sum1/2
  Reshape/1 -> Multiply/2
  Sum2/1 -> Saturation4/1  "pq_remix"
  Sum1/1 -> Saturation3/1
  PQ_Remix/1(roll_pitch_scale) -> Multiply1/2  "roll_pitch_scale"
  Saturation3/1 -> Sum2/2
  Selector/1 -> Reshape/1
  Saturation4/1 -> pq_remix_throttle/1
  Max/1 -> PQ_Remix/1(max)
  PQ_Remix/2(floating_throttle) -> Sum1/1  "floating_throttle"
  Effective_Matrix/1 -> pq_column/1
  torque_cmd/1 -> Selector/1

== system Controller/Controller/Control_Allocation/Octocopter_+/Yaw_Remix ==
  Effective_Matrix : Inport
  torque_cmd : Inport  Port=2
  pq_remix : Inport  Port=3
  Constant : Constant  Value=up_lim  OutDataTypeStr=single
  Constant1 : Constant  Value=lo_lim  OutDataTypeStr=single
  Multiply2 : Product  Multiplication=Matrix(*)  OutDataTypeStr=single
  R_Remix : MATLAB Function  TreatAsAtomicUnit=on
  Selector2 : Selector  InputPortWidth=3  IndexOptions=Index vector (dialog)  Indices=3  OutputSizes=1
  Sum3 : Sum  Inputs=|++
  Sum4 : Sum  Inputs=++|
  r_column : Selector  NumberOfDimensions=2  InputPortWidth=3  IndexOptions=Select all,Index vector (dialog)  Indices=[1:4],3  OutputSizes=1,1
  pqr_remix_throttle : Outport
  wires:
  Sum4/1 -> pqr_remix_throttle/1  "pqr_remix"
  Selector2/1 -> Multiply2/2
  Effective_Matrix/1 -> r_column/1
  torque_cmd/1 -> Selector2/1
  r_column/1 -> R_Remix/3(r_column), Multiply2/1
  Sum3/1 -> Sum4/2, R_Remix/4(motor_out)
  Multiply2/1 -> Sum3/1
  pq_remix/1 -> Sum3/2
  Constant/1 -> R_Remix/1(up_lim)
  Constant1/1 -> R_Remix/2(lo_lim)
  R_Remix/1(floating_yaw) -> Sum4/1  "floating_yaw"

== system Controller/Controller/Control_Allocation/Octocopter_+/actuator_cmd_routing ==
  throttle_cmd : Inport
  status : Inport  Port=2
  Constant : Constant  Value=zeros(8,1)  VectorParams1D=off  OutDataTypeStr=uint16
  Constant2 : Constant  Value=1000  OutDataTypeStr=uint32
  Data Type Conversion : DataTypeConversion  OutDataTypeStr=uint16
  Disarm : Constant  Value=ones(8,1)*1000  VectorParams1D=off  OutDataTypeStr=uint16
  Gain3 : Gain  Gain=1000  OutDataTypeStr=uint32
  Multiport Switch : MultiPortSwitch  DataPortForDefault=Additional data port  DiagnosticForDefault=None
  Mux1 : Mux  Inputs=2
  Reshape : Reshape  OutputDimensionality=Customize  OutputDimensions=[16,1]
  Saturation5 : Saturate  UpperLimit=1  LowerLimit=0
  Standby : Constant  Value=ones(8,1)*1150  VectorParams1D=off  OutDataTypeStr=uint16
  Sum5 : Sum  Inputs=|++
  actuator_cmd : Outport
  wires:
  Disarm/1 -> Multiport Switch/5, Multiport Switch/2
  Reshape/1 -> actuator_cmd/1
  Constant/1 -> Mux1/2
  Standby/1 -> Multiport Switch/3
  Mux1/1 -> Reshape/1
  status/1 -> Multiport Switch/1
  Multiport Switch/1 -> Mux1/1
  Sum5/1 -> Data Type Conversion/1
  Saturation5/1 -> Gain3/1
  Gain3/1 -> Sum5/1
  Constant2/1 -> Sum5/2
  throttle_cmd/1 -> Saturation5/1
  Data Type Conversion/1 -> Multiport Switch/4

== system Controller/Controller/Control_Allocation/Octocopter_x/Roll_Pitch_Remix ==
  Effective_Matrix : Inport
  torque_cmd : Inport  Port=2
  throttle_cmd : Inport  Port=3
  Constant : Constant  Value=up_lim  OutDataTypeStr=single
  Constant1 : Constant  Value=lo_lim  OutDataTypeStr=single
  Max : MinMax  Function=max
  Max1 : MinMax
  Multiply : Product  Multiplication=Matrix(*)  OutDataTypeStr=single
  Multiply1 : Product  OutDataTypeStr=single
  PQ_Remix : Subsystem
  Reshape : Reshape  OutputDimensionality=Column vector (2-D)
  Saturation3 : Saturate  UpperLimit=1  LowerLimit=0
  Saturation4 : Saturate  UpperLimit=1  LowerLimit=0
  Selector : Selector  InputPortWidth=3  IndexOptions=Index vector (dialog)  Indices=[1 2]  OutputSizes=1
  Sum : Sum  Inputs=|++
  Sum1 : Sum  Inputs=|++
  Sum2 : Sum  Inputs=|++
  pq_column : Selector  NumberOfDimensions=2  InputPortWidth=3  IndexOptions=Select all,Index vector (dialog)  Indices=[1:4],[1 2]  OutputSizes=1,1
  pq_remix_throttle : Outport
  wires:
  Multiply1/1 -> Sum2/1
  Multiply/1 -> Multiply1/1, Sum/1
  Constant1/1 -> PQ_Remix/4(lo_min)
  Sum/1 -> Max/1, Max1/1  "pq_premix"
  Max1/1 -> PQ_Remix/2(min)
  pq_column/1 -> Multiply/1
  Constant/1 -> PQ_Remix/3(up_lim)
  throttle_cmd/1 -> PQ_Remix/5(force_z_cmd), Sum/2, Sum1/2
  Reshape/1 -> Multiply/2
  Sum2/1 -> Saturation4/1  "pq_remix"
  Sum1/1 -> Saturation3/1
  PQ_Remix/1(roll_pitch_scale) -> Multiply1/2  "roll_pitch_scale"
  Saturation3/1 -> Sum2/2
  Selector/1 -> Reshape/1
  Saturation4/1 -> pq_remix_throttle/1
  Max/1 -> PQ_Remix/1(max)
  PQ_Remix/2(floating_throttle) -> Sum1/1  "floating_throttle"
  Effective_Matrix/1 -> pq_column/1
  torque_cmd/1 -> Selector/1

== system Controller/Controller/Control_Allocation/Octocopter_x/Yaw_Remix ==
  Effective_Matrix : Inport
  torque_cmd : Inport  Port=2
  pq_remix : Inport  Port=3
  Constant : Constant  Value=up_lim  OutDataTypeStr=single
  Constant1 : Constant  Value=lo_lim  OutDataTypeStr=single
  Multiply2 : Product  Multiplication=Matrix(*)  OutDataTypeStr=single
  R_Remix : MATLAB Function  TreatAsAtomicUnit=on
  Selector2 : Selector  InputPortWidth=3  IndexOptions=Index vector (dialog)  Indices=3  OutputSizes=1
  Sum3 : Sum  Inputs=|++
  Sum4 : Sum  Inputs=++|
  r_column : Selector  NumberOfDimensions=2  InputPortWidth=3  IndexOptions=Select all,Index vector (dialog)  Indices=[1:4],3  OutputSizes=1,1
  pqr_remix_throttle : Outport
  wires:
  Sum4/1 -> pqr_remix_throttle/1  "pqr_remix"
  Selector2/1 -> Multiply2/2
  Effective_Matrix/1 -> r_column/1
  torque_cmd/1 -> Selector2/1
  r_column/1 -> R_Remix/3(r_column), Multiply2/1
  Sum3/1 -> Sum4/2, R_Remix/4(motor_out)
  Multiply2/1 -> Sum3/1
  pq_remix/1 -> Sum3/2
  Constant/1 -> R_Remix/1(up_lim)
  Constant1/1 -> R_Remix/2(lo_lim)
  R_Remix/1(floating_yaw) -> Sum4/1  "floating_yaw"

== system Controller/Controller/Control_Allocation/Octocopter_x/actuator_cmd_routing ==
  throttle_cmd : Inport
  status : Inport  Port=2
  Constant : Constant  Value=zeros(8,1)  VectorParams1D=off  OutDataTypeStr=uint16
  Constant2 : Constant  Value=1000  OutDataTypeStr=uint32
  Data Type Conversion : DataTypeConversion  OutDataTypeStr=uint16
  Disarm : Constant  Value=ones(8,1)*1000  VectorParams1D=off  OutDataTypeStr=uint16
  Gain3 : Gain  Gain=1000  OutDataTypeStr=uint32
  Multiport Switch : MultiPortSwitch  DataPortForDefault=Additional data port  DiagnosticForDefault=None
  Mux1 : Mux  Inputs=2
  Reshape : Reshape  OutputDimensionality=Customize  OutputDimensions=[16,1]
  Saturation5 : Saturate  UpperLimit=1  LowerLimit=0
  Standby : Constant  Value=ones(8,1)*1150  VectorParams1D=off  OutDataTypeStr=uint16
  Sum5 : Sum  Inputs=|++
  actuator_cmd : Outport
  wires:
  Disarm/1 -> Multiport Switch/5, Multiport Switch/2
  Reshape/1 -> actuator_cmd/1
  Constant/1 -> Mux1/2
  Standby/1 -> Multiport Switch/3
  Mux1/1 -> Reshape/1
  status/1 -> Multiport Switch/1
  Multiport Switch/1 -> Mux1/1
  Sum5/1 -> Data Type Conversion/1
  Saturation5/1 -> Gain3/1
  Gain3/1 -> Sum5/1
  Constant2/1 -> Sum5/2
  throttle_cmd/1 -> Saturation5/1
  Data Type Conversion/1 -> Multiport Switch/4

== system Controller/Controller/Control_Allocation/Quadcopter_+/Roll_Pitch_Remix ==
  Effective_Matrix : Inport
  torque_cmd : Inport  Port=2
  throttle_cmd : Inport  Port=3
  Constant : Constant  Value=up_lim  OutDataTypeStr=single
  Constant1 : Constant  Value=lo_lim  OutDataTypeStr=single
  Max : MinMax  Function=max
  Max1 : MinMax
  Multiply : Product  Multiplication=Matrix(*)  OutDataTypeStr=single
  Multiply1 : Product  OutDataTypeStr=single
  PQ_Remix : Subsystem
  Reshape : Reshape  OutputDimensionality=Column vector (2-D)
  Saturation3 : Saturate  UpperLimit=1  LowerLimit=0
  Saturation4 : Saturate  UpperLimit=1  LowerLimit=0
  Selector : Selector  InputPortWidth=3  IndexOptions=Index vector (dialog)  Indices=[1 2]  OutputSizes=1
  Sum : Sum  Inputs=|++
  Sum1 : Sum  Inputs=|++
  Sum2 : Sum  Inputs=|++
  pq_column : Selector  NumberOfDimensions=2  InputPortWidth=3  IndexOptions=Index vector (dialog),Index vector (dialog)  Indices=[1:4],[1 2]  OutputSizes=1,1
  pq_remix_throttle : Outport
  wires:
  Multiply1/1 -> Sum2/1
  Multiply/1 -> Multiply1/1, Sum/1
  Constant1/1 -> PQ_Remix/4(lo_min)
  Sum/1 -> Max/1, Max1/1  "pq_premix"
  Max1/1 -> PQ_Remix/2(min)
  pq_column/1 -> Multiply/1
  Constant/1 -> PQ_Remix/3(up_lim)
  throttle_cmd/1 -> PQ_Remix/5(force_z_cmd), Sum/2, Sum1/2
  Reshape/1 -> Multiply/2
  Sum2/1 -> Saturation4/1  "pq_remix"
  Sum1/1 -> Saturation3/1
  PQ_Remix/1(roll_pitch_scale) -> Multiply1/2  "roll_pitch_scale"
  Saturation3/1 -> Sum2/2
  Selector/1 -> Reshape/1
  Saturation4/1 -> pq_remix_throttle/1
  Max/1 -> PQ_Remix/1(max)
  PQ_Remix/2(floating_throttle) -> Sum1/1  "floating_throttle"
  Effective_Matrix/1 -> pq_column/1
  torque_cmd/1 -> Selector/1

== system Controller/Controller/Control_Allocation/Quadcopter_+/Yaw_Remix ==
  Effective_Matrix : Inport
  torque_cmd : Inport  Port=2
  pq_remix : Inport  Port=3
  Constant : Constant  Value=up_lim  OutDataTypeStr=single
  Constant1 : Constant  Value=lo_lim  OutDataTypeStr=single
  Multiply2 : Product  Multiplication=Matrix(*)  OutDataTypeStr=single
  R_Remix : MATLAB Function  TreatAsAtomicUnit=on
  Selector2 : Selector  InputPortWidth=3  IndexOptions=Index vector (dialog)  Indices=3  OutputSizes=1
  Sum3 : Sum  Inputs=|++
  Sum4 : Sum  Inputs=++|
  r_column : Selector  NumberOfDimensions=2  InputPortWidth=3  IndexOptions=Index vector (dialog),Index vector (dialog)  Indices=[1:4],3  OutputSizes=1,1
  pqr_remix_throttle : Outport
  wires:
  Sum4/1 -> pqr_remix_throttle/1  "pqr_remix"
  Selector2/1 -> Multiply2/2
  Effective_Matrix/1 -> r_column/1
  torque_cmd/1 -> Selector2/1
  r_column/1 -> R_Remix/3(r_column), Multiply2/1
  Sum3/1 -> Sum4/2, R_Remix/4(motor_out)
  Multiply2/1 -> Sum3/1
  pq_remix/1 -> Sum3/2
  Constant/1 -> R_Remix/1(up_lim)
  Constant1/1 -> R_Remix/2(lo_lim)
  R_Remix/1(floating_yaw) -> Sum4/1  "floating_yaw"

== system Controller/Controller/Control_Allocation/Quadcopter_+/actuator_cmd_routing ==
  throttle_cmd : Inport
  status : Inport  Port=2
  Constant : Constant  Value=zeros(12,1)  VectorParams1D=off  OutDataTypeStr=uint16
  Constant2 : Constant  Value=1000  OutDataTypeStr=uint32
  Data Type Conversion : DataTypeConversion  OutDataTypeStr=uint16
  Disarm : Constant  Value=ones(4,1)*1000  VectorParams1D=off  OutDataTypeStr=uint16
  Gain3 : Gain  Gain=1000  OutDataTypeStr=uint32
  Multiport Switch : MultiPortSwitch  DataPortForDefault=Additional data port  DiagnosticForDefault=None
  Mux1 : Mux  Inputs=2
  Reshape : Reshape  OutputDimensionality=Customize  OutputDimensions=[16,1]
  Saturation5 : Saturate  UpperLimit=1  LowerLimit=0
  Standby : Constant  Value=ones(4,1)*1150  VectorParams1D=off  OutDataTypeStr=uint16
  Sum5 : Sum  Inputs=|++
  actuator_cmd : Outport
  wires:
  Disarm/1 -> Multiport Switch/5, Multiport Switch/2
  Reshape/1 -> actuator_cmd/1
  Constant/1 -> Mux1/2
  Standby/1 -> Multiport Switch/3
  Mux1/1 -> Reshape/1
  status/1 -> Multiport Switch/1
  Multiport Switch/1 -> Mux1/1
  Sum5/1 -> Data Type Conversion/1
  Saturation5/1 -> Gain3/1
  Gain3/1 -> Sum5/1
  Constant2/1 -> Sum5/2
  throttle_cmd/1 -> Saturation5/1
  Data Type Conversion/1 -> Multiport Switch/4
